simulink model "vdynblksskidpad_final"  (R2026b)
settings: Solver=ode23t  StopTime=inf  RelTol=5e-3
model workspace (MAT data in the model file):
  Eng : object (value not decoded)
  Nmtr = 11.5
  StartupTrim : object (value not decoded)
  SteerLim = 60
  TrackPoints = [-15 -12 -9 -6 -3 5.58745102111e-16 2.81978007367 5.36354042717 7.38228007367 8.67839071119 9.125 8.67839071119 ... (270 elements, 90x3)]
  Trans : object (value not decoded)
  Ts = 0.02
  VEH : object (value not decoded)
values from neighbouring files (symbols this model uses):
  n = size(e.Data,2)    [plot_skidpad_signals.m]
  z = tsMatrix(out.diagWheel.z)    [skidpad_settle_start.m]
symbols that are objects in the model workspace (value not decoded): Eng, StartupTrim, Trans, VEH
undefined symbols (not defined in the file or in its folder): BdyFrm, InertFrm, magnitude
libraries: autolibsharedcoupling x11, simulink x8, sim3dlib x7, autolibshareddiff x5, autolibutils x4, sim3dautolib x3, vehdynlibtirecommon x3, sharedtransform x3, vehdynlibdriver x2, vehdynlibsteering x2, vehdynlibeom x2, vehdynlibviscommon x2
(part 4 of 5)

== system vdynblksskidpad_final/Formula Student Vehicle/Simulink Physics - 7DOF/Powertrain & Driveline/Powertrain/4EM Powertrain/Mapped Motors ==
  BattVolt : Inport  Partition=on  PartitionDimension=1  PartitionWidth=1  PartitionOffset=0
  MtrSpd : Inport  Port=2  Partition=on  PartitionDimension=1  PartitionWidth=1  PartitionOffset=0
  TrqCmd : Inport  Port=3  Partition=on  PartitionDimension=1  PartitionWidth=1  PartitionOffset=0
  For Each : ForEach  DisableCoverage=on
  Mapped Motor : autolibmappedmotor/Mapped Motor  w_Tmax_bp_ext=[-800;-750;-375;0;375;750;800]  Tmax_w_V_ext=[0 0 0;0.07 0.07 0.07;0.08 0.08 0.08;0.09 0.09 0.09;0.08 0.08 0.08;0.07 0.07 0.07;0 0 0]  w_Tmin_bp_ext=[-800;-750;-375;0;375;750;800]  Tmin_w_V_ext=[0 0 0;-0.07 -0.07 -0.07;-0.08 -0.08 -0.08;-0.09 -0.09 -0.09;-0.08 -0.08 -0.08;-0.07 -0.07 -0.07;0 0 0]  port_config=Speed  param_by=Maximum torque and power  w_t=[0 954.93 1909.86 3819.72 4774.65 5729.58 7639.44 9549.30 11459.16 13369.02 15278.88 17188.74 19098.59 20000]*pi/30  T_t=[40 40 40 40 40 33.33 25.00 20.00 16.67 14.29 12.50 11.11 10.00 9.55]  torque_max=31.6  power_max=35000  SpreadsheetTqLimitsFileName=MotorCalibrationImportData.xlsx  Tmax_w_V=[0.09 0.09 0.09;0.08 0.08 0.08;0.07 0.07 0.07;0 0 0]  w_Tmax_bp=[ 0 375 750 800 ]  V_Tmax_bp=[500 750 900]  Tmin_w_V=[-0.09 -0.09 -0.09;-0.08 -0.08 -0.08;-0.07 -0.07 -0.07;0 0 0]  w_Tmin_bp=[ 0 375 750 800 ]  V_Tmin_bp=[500 750 900]  Tc=.02  param_loss=Single efficiency measurement  SpreadsheetLossFileName=MotorCalibrationImportData.xlsx  SpreadsheetEffFileName=MotorCalibrationImportData.xlsx  eff=96  w_eff=4000  T_eff=40  Piron=400  Pbase=0  w_eff_bp=[-8000 -4000 0 4000 8000]  T_eff_bp=[0 0.03 0.06 0.09]  Temp_eff_bp=[233.15 293.15 373.15]  V_eff_bp=[500 700 900]  losses_table=[1.49 1.67 2.21 3.10; 0.42 0.69 1.14 2.03; 0.06 0.24 0.78 1.68; 0.42 0.69 1.14 2.03; 1.49 1.67 2.21 3.10]  losses_table_3d=cat(3,1.05*[1.49 1.67 2.21 3.10; 0.42 0.69 1.14 2.03; 0.06 0.24 0.78 1.68; 0.42 0.69 1.14 2.03; 1.49 1.67 2.21 3.10],[1.49 1.67 2.21 3.10; 0.42 0.69 1.14 2.03; 0.06 0.24 0.78 1.68; 0.42 0.69 1.14 2.03; 1.49 1.67 2.21 3.10],1.03*[1.49 1.67 2.21 3.10; 0.42 0.69 1.14 2.03; 0.06 0.24 0.78 1.68; 0.42 0.69 1.14 2.03; 1.49 1.67 2.21 3.10])  losses_table_4d=cat(4,cat(3,[1.5645 0.441 0.063 0.441 1.5645;1.7535 0.7245 0.252 0.7245 1.7535;2.3205 1.197 0.819 1.197 2.3205;3.255 2.1315 1.764 2.1315 3.255],[1.5645 0.441 0.063 0.441 1.5645;1.7535 0.7245 0.252 0.7245 1.7535;2.3205 1.197 0.819 1.197 2.3205;3.255 2.1315 1.764 2.1315 3.255],[1.5645 0.441 0.063 0.441 1.5645;1.7535 0.7245 0.252 0.7245 1.7535;2.3205 1.197 0.819 1.197 2.3205;3.255 2.1315 1.764 2.1315 3.255]),cat(3,[1.49 0.42 0.06 0.42 1.49;1.67 0.69 0.24 0.69 1.67;2.21 1.14 0.78 1.14 2.21;3.1 2.03 1.68 2.03 3.1],[1.49 0.42 0.06 0.42 1.49;1.67 0.69 0.24 0.69 1.67;2.21 1.14 0.78 1.14 2.21;3.1 2.03 1.68 2.03 3.1],[1.49 0.42 0.06 0.42 1.49;1.67 0.69 0.24 0.69 1.67;2.21 1.14 0.78 1.14 2.21;3.1 2.03 1.68 2.03 3.1]),cat(3,[1.5347 0.4326 0.0618 0.4326 1.5347;1.7201 0.7107 0.2472 0.7107 1.7201;2.2763 1.1742 0.8034 1.1742 2.2763;3.193 2.0909 1.7304 2.0909 3.193],[1.5347 0.4326 0.0618 0.4326 1.5347;1.7201 0.7107 0.2472 0.7107 1.7201;2.2763 1.1742 0.8034 1.1742 2.2763;3.193 2.0909 1.7304 2.0909 3.193],[1.5347 0.4326 0.0618 0.4326 1.5347;1.7201 0.7107 0.2472 0.7107 1.7201;2.2763 1.1742 0.8034 1.1742 2.2763;3.193 2.0909 1.7304 2.0909 3.193]))  efficiency_table=[95 95 95 95; 95 95 95 95; 95 95 95 95; 95 95 95 95; 95 95 95 95]  efficiency_table_3d=cat(3,90*ones(5,4),95*ones(5,4),92*ones(5,4))  efficiency_table_4d=cat(4,cat(3,90*ones(5,4)',90*ones(5,4)',90*ones(5,4)'),cat(3,95*ones(5,4)',95*ones(5,4)',95*ones(5,4)'),cat(3,92*ones(5,4)',92*ones(5,4)',92*ones(5,4)'))  J=5e-6  b=1e-5  omega_o=0  T_t_extended=[0 15.4 17.6 20.9 17.6 15.4 0]  w_t_extended=[-8000 -7500 -3750 0 3750 7500 8000]  KLossIron=0  KLossCopper=0  x_w_eff_vec=[-8000 -4000 0 4000 8000]  x_T_eff_vec=[-0.09 -0.06 -0.03 0 0.03 0.06 0.09]  x_tmp_eff_vec=[233.15 293.15 373.15]  x_V_eff_vec=[500 700 900]  x_losses_mat=[3.1 2.21 1.67 1.49 1.67 2.21 3.1;2.03 1.14 0.69 0.42 0.69 1.14 2.03;1.68 0.78 0.24 0.06 0.24 0.78 1.68;2.03 1.14 0.69 0.42 0.69 1.14 2.03;3.1 2.21 1.67 1.49 1.67 2.21 3.1]  x_losses_mat_3d=cat(3,[3.255 2.3205 1.7535 1.5645 1.7535 2.3205 3.255;2.1315 1.197 0.7245 0.441 0.7245 1.197 2.1315;1.764 0.819 0.252 0.063 0.252 0.819 1.764;2.1315 1.197 0.7245 0.441 0.7245 1.197 2.1315;3.255 2.3205 1.7535 1.5645 1.7535 2.3205 3.255],[3.1 2.21 1.67 1.49 1.67 2.21 3.1;2.03 1.14 0.69 0.42 0.69 1.14 2.03;1.68 0.78 0.24 0.06 0.24 0.78 1.68;2.03 1.14 0.69 0.42 0.69 1.14 2.03;3.1 2.21 1.67 1.49 1.67 2.21 3.1],[3.193 2.2763 1.7201 1.5347 1.7201 2.2763 3.193;2.0909 1.1742 0.7107 0.4326 0.7107 1.1742 2.0909;1.7304 0.8034 0.2472 0.0618 0.2472 0.8034 1.7304;2.0909 1.1742 0.7107 0.4326 0.7107 1.1742 2.0909;3.193 2.2763 1.7201 1.5347 1.7201 2.2763 3.193])  x_losses_mat_4d=cat(4,cat(3,[1.5645 0.441 0.063 0.441 1.5645;1.7535 0.7245 0.252 0.7245 1.7535;2.3205 1.197 0.819 1.197 2.3205;3.255 2.1315 1.764 2.1315 3.255],[1.5645 0.441 0.063 0.441 1.5645;1.7535 0.7245 0.252 0.7245 1.7535;2.3205 1.197 0.819 1.197 2.3205;3.255 2.1315 1.764 2.1315 3.255],[1.5645 0.441 0.063 0.441 1.5645;1.7535 0.7245 0.252 0.7245 1.7535;2.3205 1.197 0.819 1.197 2.3205;3.255 2.1315 1.764 2.1315 3.255]),cat(3,[1.49 0.42 0.06 0.42 1.49;1.67 0.69 0.24 0.69 1.67;2.21 1.14 0.78 1.14 2.21;3.1 2.03 1.68 2.03 3.1],[1.49 0.42 0.06 0.42 1.49;1.67 0.69 0.24 0.69 1.67;2.21 1.14 0.78 1.14 2.21;3.1 2.03 1.68 2.03 3.1],[1.49 0.42 0.06 0.42 1.49;1.67 0.69 0.24 0.69 1.67;2.21 1.14 0.78 1.14 2.21;3.1 2.03 1.68 2.03 3.1]),cat(3,[1.5347 0.4326 0.0618 0.4326 1.5347;1.7201 0.7107 0.2472 0.7107 1.7201;2.2763 1.1742 0.8034 1.1742 2.2763;3.193 2.0909 1.7304 2.0909 3.193],[1.5347 0.4326 0.0618 0.4326 1.5347;1.7201 0.7107 0.2472 0.7107 1.7201;2.2763 1.1742 0.8034 1.1742 2.2763;3.193 2.0909 1.7304 2.0909 3.193],[1.5347 0.4326 0.0618 0.4326 1.5347;1.7201 0.7107 0.2472 0.7107 1.7201;2.2763 1.1742 0.8034 1.1742 2.2763;3.193 2.0909 1.7304 2.0909 3.193]))  CalLossMapData={}  CalLossWithTempMapData={}  aMode=2  RefBlkName='autolibmappedmotor/Mapped Motor'
      settings: LibrarySourceBlock=vdynlib/Powertrain/Propulsion/Mapped Motor
  Power and Torque Management : Subsystem
  Terminator : Terminator
  MtrTrq : Outport  ConcatenationDimension=1
  BattCurr : Outport  Port=2  ConcatenationDimension=1
  TrqLimCmd : Outport  Port=3  ConcatenationDimension=1
  wires:
  Mapped Motor/2 -> BattCurr/1
  TrqCmd/1 -> Power and Torque Management/2(TrqCmd)
  Mapped Motor/1 -> Terminator/1
  MtrSpd/1 -> Power and Torque Management/1(MtrSpd), Mapped Motor/2
  Mapped Motor/3 -> MtrTrq/1
  Power and Torque Management/1(TrqLimCmd) -> TrqLimCmd/1, Mapped Motor/3
  BattVolt/1 -> Mapped Motor/1

== system vdynblksskidpad_final/Formula Student Vehicle/Simulink Physics - 7DOF/Powertrain & Driveline/Powertrain/ICE Powertrain/Transmission ==
  EngTrq : Inport
  GearCmd : Inport  Port=2
  PropShftSpd : Inport  Port=3
  Ideal : Subsystem  VariantControl=0
  EngSpd : Outport  VectorParamsAs1DForOutWhenUnconnected=off
  Info : Outport  Port=2  VectorParamsAs1DForOutWhenUnconnected=off
  DrvShfTrq : Outport  Port=3  VectorParamsAs1DForOutWhenUnconnected=off

== system vdynblksskidpad_final/Visualization/3D Visualization/Enabled/3D Visualization/Ground Following/Annotations ==
  VehFdbk : Inport
  Disabled : Subsystem  VariantControl=annotOn==0
  Enabled : Subsystem  VariantControl=annotOn==1

== system vdynblksskidpad_final/Visualization/3D Visualization/Enabled/3D Visualization/Ground Following/Path ==
  VehFdbk : Inport
  Disabled : Subsystem  VariantControl=pathOn==0
  Enabled : Subsystem  VariantControl=pathOn==1

== system vdynblksskidpad_final/Visualization/3D Visualization/Enabled/3D Visualization/Physical Vehicle/Annotations ==
  VehFdbk : Inport
  Disabled : Subsystem  VariantControl=annotOn==0
  Enabled : Subsystem  VariantControl=annotOn==1

== system vdynblksskidpad_final/Visualization/3D Visualization/Enabled/3D Visualization/Physical Vehicle/Path ==
  VehFdbk : Inport
  Disabled : Subsystem  VariantControl=pathOn==0
  Enabled : Subsystem  VariantControl=pathOn==1

== system vdynblksskidpad_final/Visualization/3D Visualization/Enabled/3D Visualization/Simulation 3D Vehicle/Annotations ==
  VehFdbk : Inport
  Disabled : Subsystem  VariantControl=annotOn==0
  Enabled : Subsystem  VariantControl=annotOn==1

== system vdynblksskidpad_final/Visualization/3D Visualization/Enabled/3D Visualization/Simulation 3D Vehicle/Part Rotation Concatenation ==
  Body Roll : Inport
  Body Ptich : Inport  Port=2
  Body Yaw : Inport  Port=3
  WheelFrontLeft Pitch : Inport  Port=4
  WheelFrontRight Pitch : Inport  Port=5
  WheelRearLeft Pitch : Inport  Port=6
  WheelRearRight Ptich : Inport  Port=7
  WheelFrontLeft Roll : Inport  Port=8
  WheelFrontRight Roll : Inport  Port=9
  WheelRearLeft Roll : Inport  Port=10
  WheelRearRight Roll : Inport  Port=11
  WheelFrontLeft Yaw : Inport  Port=12
  WheelFrontRight Yaw : Inport  Port=13
  WheelRearLeft Yaw : Inport  Port=14
  WheelRearRight Yaw : Inport  Port=15
  AllParts : Concatenate  NumInputs=5  Mode=Multidimensional array
  Body : Concatenate  NumInputs=3  Mode=Multidimensional array  ConcatenateDimension=2
  WheelFrontLeft : Concatenate  NumInputs=3  Mode=Multidimensional array  ConcatenateDimension=2
  WheelFrontRight : Concatenate  NumInputs=3  Mode=Multidimensional array  ConcatenateDimension=2
  WheelRearLeft : Concatenate  NumInputs=3  Mode=Multidimensional array  ConcatenateDimension=2
  WheelRearRight : Concatenate  NumInputs=3  Mode=Multidimensional array  ConcatenateDimension=2
  ConcatOut : Outport  VectorParamsAs1DForOutWhenUnconnected=off
  wires:
  Body Yaw/1 -> Body/3
  WheelFrontLeft Yaw/1 -> WheelFrontLeft/3
  WheelFrontLeft/1 -> AllParts/2
  Body/1 -> AllParts/1
  WheelRearLeft/1 -> AllParts/4
  WheelFrontRight/1 -> AllParts/3
  WheelRearRight Yaw/1 -> WheelRearRight/3
  WheelRearLeft Yaw/1 -> WheelRearLeft/3
  AllParts/1 -> ConcatOut/1
  WheelRearRight/1 -> AllParts/5
  WheelFrontRight Yaw/1 -> WheelFrontRight/3
  Body Ptich/1 -> Body/2
  Body Roll/1 -> Body/1
  WheelFrontLeft Pitch/1 -> WheelFrontLeft/2
  WheelFrontLeft Roll/1 -> WheelFrontLeft/1
  WheelFrontRight Pitch/1 -> WheelFrontRight/2
  WheelFrontRight Roll/1 -> WheelFrontRight/1
  WheelRearLeft Pitch/1 -> WheelRearLeft/2
  WheelRearLeft Roll/1 -> WheelRearLeft/1
  WheelRearRight Ptich/1 -> WheelRearRight/2
  WheelRearRight Roll/1 -> WheelRearRight/1

== system vdynblksskidpad_final/Visualization/3D Visualization/Enabled/3D Visualization/Simulation 3D Vehicle/Part Translation Concatenation ==
  BodyX : Inport
  BodyY : Inport  Port=2
  BodyZ : Inport  Port=3
  WheelFrontLeftX : Inport  Port=4
  WheelFrontRightX : Inport  Port=5
  WheelRearLeftX : Inport  Port=6
  WheelRearRightX : Inport  Port=7
  WheelFrontLeftY : Inport  Port=8
  WheelFrontRightY : Inport  Port=9
  WheelRearLeftY : Inport  Port=10
  WheelRearRightY : Inport  Port=11
  WheelFrontLeftZ : Inport  Port=12
  WheelFrontRightZ : Inport  Port=13
  WheelRearLeftZ : Inport  Port=14
  WheelRearRightZ : Inport  Port=15
  AllParts : Concatenate  NumInputs=5  Mode=Multidimensional array
  Body : Concatenate  NumInputs=3  Mode=Multidimensional array  ConcatenateDimension=2
  WheelFrontLeft : Concatenate  NumInputs=3  Mode=Multidimensional array  ConcatenateDimension=2
  WheelFrontRight : Concatenate  NumInputs=3  Mode=Multidimensional array  ConcatenateDimension=2
  WheelRearLeft : Concatenate  NumInputs=3  Mode=Multidimensional array  ConcatenateDimension=2
  WheelRearRight : Concatenate  NumInputs=3  Mode=Multidimensional array  ConcatenateDimension=2
  ConcatOut : Outport  VectorParamsAs1DForOutWhenUnconnected=off
  wires:
  BodyX/1 -> Body/1
  BodyZ/1 -> Body/3
  WheelFrontLeftX/1 -> WheelFrontLeft/1
  WheelFrontLeftZ/1 -> WheelFrontLeft/3
  WheelFrontLeftY/1 -> WheelFrontLeft/2
  BodyY/1 -> Body/2
  WheelFrontLeft/1 -> AllParts/2
  WheelRearRightX/1 -> WheelRearRight/1
  Body/1 -> AllParts/1
  WheelRearLeft/1 -> AllParts/4
  WheelFrontRight/1 -> AllParts/3
  WheelRearRightZ/1 -> WheelRearRight/3
  WheelFrontRightY/1 -> WheelFrontRight/2
  WheelFrontRightX/1 -> WheelFrontRight/1
  WheelRearRightY/1 -> WheelRearRight/2
  WheelRearLeftZ/1 -> WheelRearLeft/3
  AllParts/1 -> ConcatOut/1
  WheelRearLeftY/1 -> WheelRearLeft/2
  WheelRearRight/1 -> AllParts/5
  WheelRearLeftX/1 -> WheelRearLeft/1
  WheelFrontRightZ/1 -> WheelFrontRight/3

== system vdynblksskidpad_final/Visualization/3D Visualization/Enabled/3D Visualization/Simulation 3D Vehicle/Path ==
  VehFdbk : Inport
  Disabled : Subsystem  VariantControl=pathOn==0
  Enabled : Subsystem  VariantControl=pathOn==1

== system vdynblksskidpad_final/Visualization/3D Visualization/Enabled/3D Visualization/Simulation 3D Vehicle/Scale ==
  Constant{1..12,17,32..33} (15 alike) : Constant  OutDataTypeStr=single
  PartConcatenation : Subsystem
  ScaleOut : Outport  VectorParamsAs1DForOutWhenUnconnected=off
  wires:
  Constant10/1 -> PartConcatenation/15(WheelRearRightZ)
  Constant9/1 -> PartConcatenation/14(WheelRearRightY)
  Constant11/1 -> PartConcatenation/13(WheelRearRightX)
  Constant7/1 -> PartConcatenation/12(WheelRearLeftZ)
  Constant6/1 -> PartConcatenation/11(WheelRearLeftY)
  Constant8/1 -> PartConcatenation/10(WheelRearLeftX)
  Constant4/1 -> PartConcatenation/9(WheelFrontRightZ)
  Constant3/1 -> PartConcatenation/8(WheelFrontRightY)
  Constant5/1 -> PartConcatenation/7(WheelFrontRightX)
  Constant2/1 -> PartConcatenation/6(WheelFrontLeftZ)
  Constant1/1 -> PartConcatenation/5(WheelFrontLeftY)
  Constant33/1 -> PartConcatenation/4(WheelFrontLeftX)
  Constant32/1 -> PartConcatenation/3(BodyZ)
  Constant17/1 -> PartConcatenation/2(BodyY)
  Constant12/1 -> PartConcatenation/1(BodyX)
  PartConcatenation/1(ConcatOut) -> ScaleOut/1

== system vdynblksskidpad_final/Formula Student Vehicle/Simulink Physics - 7DOF/Powertrain & Driveline/Powertrain/4EM Powertrain/Mapped Motors/Power and Torque Management ==
  MtrSpd : Inport
  TrqCmd : Inport  Port=2
  Abs1 : Abs  ZeroCross=off  SaturateOnIntegerOverflow=off
  Abs2 : Abs  ZeroCross=off  SaturateOnIntegerOverflow=off
  Divide1 : Product  Inputs=*/
  MaxPwr : Constant  Value=20e3
  Product : Product
  PwrLimCorner : Gain  Gain=2
  Saturation Dynamic : sl_discontinuities/Saturation Dynamic  OutMin=[]  OutMax=[]  OutDataTypeStr=Inherit: Same as second input  OutDataType=fixdt(1, 16)  OutScaling=2^-10  DoSatur=off
  Saturation2 : Saturate  UpperLimit=inf  LowerLimit=1  ZeroCross=off
  Saturation3 : Saturate  UpperLimit=40  LowerLimit=0  ZeroCross=off
  Subtract : Sum  Inputs=+-
  Transfer Fcn : TransferFcn  Denominator=[0.1 1]
  Unary Minus : UnaryMinus
  div0protect : autolibutils/div0protect - poly  thresh=1  ZeroCross=off  ZeroCross1=on  aMode=2
  TrqLimCmd : Outport
  wires:
  Product/1 -> Abs1/1
  MtrSpd/1 -> Product/2, Abs2/1
  MaxPwr/1 -> PwrLimCorner/1
  Abs1/1 -> Subtract/2
  Saturation2/1 -> Divide1/1  "PwrLim"
  Unary Minus/1 -> Saturation Dynamic/3
  Divide1/1 -> Saturation3/1
  Abs2/1 -> div0protect/1
  div0protect/1 -> Divide1/2
  TrqCmd/1 -> Saturation Dynamic/2
  Saturation3/1 -> Saturation Dynamic/1, Unary Minus/1  "AxlTrqLim"
  Subtract/1 -> Saturation2/1
  Saturation Dynamic/1 -> TrqLimCmd/1, Transfer Fcn/1
  Transfer Fcn/1 -> Product/1
  PwrLimCorner/1 -> Subtract/1

== system vdynblksskidpad_final/Formula Student Vehicle/Simulink Physics - 7DOF/Powertrain & Driveline/Powertrain/ICE Powertrain/Transmission/Ideal ==
  GearCmd : Inport
  EngTrq : Inport  Port=2
  PropShftSpd : Inport  Port=3
  Ideal Fixed Gear Transmission : autolibsharedtransfixedgear/Ideal Fixed Gear Transmission  VariantControl=0  TransEffModelPopup=Gear only  gearInterp=Linear point-slope  G=Trans.GearNums  Trq_bpts=[25, 50, 75, 100, 150, 200, 250]  omega_bpts=[52.4 78.5 105 131 157 183 209 262 314 419 524]  Temp_bpts=[313 358]  N=Trans.GearRatios  Jout=Trans.Inertias  bout=Trans.DampingCoeffs  eta=Trans.Efficiencies  eta_tbl=reshape([0.53 0.71 0.77 0.79 0.82 0.82 0.82 0.5 0.7 0.77 0.79 0.82 0.82 0.82 0.54 0.72 0.78 0.81 0.83 0.82 0.82 0.56 0.73 0.79 0.81 0.84 0.82 0.82 0.58 0.74 0.79 0.82 0.84 0.82 0.82 0.57 0.74 0.79 0.82 0.84 0.82 0.82 0.58 0.74 0.79 0.82 0.84 0.82 0.82 0.58 0.74 0.79 0.82 0.84 0.82 0.82 0.57 0.74 0.8 0.82 0.85 0.82 0.82 0.55 0.73 0.78 0.81 0.84 0.82 0.82 0.51 0.71 0.77 0.81 0.84 0.82 0.82 0.53 0.71 0.77 0.79 0.82 0.82 0.82 0.5 0.7 0.77 0.79 0.82 0.82 0.82 0.54 0.72 0.78 0.81 0.83 0.82 0.82 0.56 0.73 0.79 0.81 0.84 0.82 0.82 0.58 0.74 0.79 0.82 0.84 0.82 0.82 0.57 0.74 0.79 0.82 0.84 0.82 0.82 0.58 0.74 0.79 0.82 0.84 0.82 0.82 0.58 0.74 0.79 0.82 0.84 0.82 0.82 0.57 0.74 0.8 0.82 0.85 0.82 0.82 0.55 0.73 0.78 0.81 0.84 0.82 0.82 0.51 0.71 0.77 0.81 0.84 0.82 0.82 0.53 0.71 0.77 0.79 0.82 0.82 0.82 0.5 0.7 0.77 0.79 0.82 0.82 0.82 0.54 0.72 0.78 0.81 0.83 0.82 0.82 0.56 0.73 0.79 0.81 0.84 0.82 0.82 0.58 0.74 0.79 0.82 0.84 0.82 0.82 0.57 0.74 0.79 0.82 0.84 0.82 0.82 0.58 0.74 0.79 0.82 0.84 0.82 0.82 0.58 0.74 0.79 0.82 0.84 0.82 0.82 0.57 0.74 0.8 0.82 0.85 0.82 0.82 0.55 0.73 0.78 0.81 0.84 0.82 0.82 0.51 0.71 0.77 0.81 0.84 0.82 0.82 0.7 0.79 0.82 0.83 0.84 0.84 0.84 0.63 0.76 0.8 0.82 0.83 0.84 0.84 0.58 0.74 0.79 0.81 0.83 0.84 0.84 0.58 0.74 0.79 0.81 0.83 0.84 0.84 0.58 0.74 0.79 0.81 0.84 0.84 0.84 0.57 0.73 0.78 0.81 0.84 0.85 0.84 0.57 0.73 0.79 0.81 0.84 0.85 0.84 0.56 0.73 0.78 0.81 0.83 0.85 0.84 0.55 0.73 0.78 0.81 0.84 0.85 0.84 0.52 0.71 0.77 0.8 0.83 0.85 0.84 0.48 0.69 0.76 0.79 0.83 0.84 0.84 0.64 0.76 0.8 0.81 0.83 0.84 0.84 0.56 0.73 0.78 0.8 0.83 0.84 0.84 0.54 0.71 0.77 0.8 0.82 0.84 0.84 0.53 0.71 0.77 0.8 0.83 0.84 0.84 0.51 0.71 0.77 0.8 0.83 0.84 0.85 0.52 0.7 0.77 0.8 0.83 0.84 0.85 0.51 0.71 0.76 0.79 0.83 0.84 0.85 0.5 0.69 0.76 0.79 0.82 0.84 0.85 0.45 0.68 0.75 0.78 0.82 0.84 0.85 0.43 0.67 0.74 0.78 0.81 0.83 0.84 0.38 0.63 0.71 0.75 0.8 0.82 0.83 0.65 0.79 0.84 0.85 0.88 0.89 0.89 0.56 0.75 0.81 0.83 0.86 0.88 0.89 0.52 0.72 0.79 0.83 0.86 0.88 0.88 0.51 0.72 0.79 0.83 0.86 0.88 0.89 0.49 0.71 0.78 0.82 0.86 0.88 0.89 0.47 0.7 0.78 0.82 0.86 0.87 0.88 0.45 0.69 0.77 0.81 0.85 0.87 0.88 0.4 0.67 0.75 0.8 0.84 0.86 0.88 0.3 0.64 0.73 0.78 0.83 0.86 0.87 0.17 0.55 0.67 0.73 0.8 0.83 0.85 0.089 0.45 0.61 0.69 0.77 0.81 0.83 0.61 0.75 0.82 0.84 0.87 0.87 0.88 0.54 0.73 0.8 0.82 0.86 0.87 0.88 0.51 0.71 0.79 0.82 0.86 0.87 0.88 0.52 0.72 0.79 0.82 0.86 0.87 0.89 0.52 0.72 0.8 0.83 0.86 0.88 0.89 0.53 0.72 0.79 0.82 0.86 0.87 0.89 0.5 0.7 0.78 0.82 0.86 0.88 0.88 0.46 0.69 0.77 0.81 0.85 0.87 0.88 0.4 0.67 0.75 0.8 0.83 0.86 0.88 0.33 0.64 0.73 0.78 0.83 0.85 0.87 0.33 0.64 0.73 0.78 0.83 0.85 0.87 0.78 0.85 0.87 0.88 0.89 0.89 0.89 0.73 0.83 0.86 0.88 0.89 0.89 0.89 0.72 0.83 0.86 0.88 0.89 0.89 0.89 0.72 0.83 0.87 0.89 0.9 0.89 0.89 0.72 0.83 0.87 0.88 0.9 0.89 0.89 0.71 0.83 0.87 0.88 0.9 0.89 0.89 0.71 0.83 0.86 0.88 0.9 0.89 0.89 0.7 0.82 0.86 0.88 0.9 0.89 0.89 0.69 0.82 0.86 0.88 0.9 0.89 0.89 0.67 0.81 0.86 0.88 0.9 0.89 0.89 0.63 0.79 0.85 0.87 0.89 0.89 0.89 0.78 0.85 0.87 0.88 0.89 0.89 0.89 0.73 0.83 0.86 0.88 0.89 0.89 0.89 0.72 0.83 0.86 0.88 0.89 0.89 0.89 0.72 0.83 0.87 0.89 0.9 0.89 0.89 0.72 0.83 0.87 0.88 0.9 0.89 0.89 0.71 0.83 0.87 0.88 0.9 0.89 0.89 0.71 0.83 0.86 0.88 0.9 0.89 0.89 0.7 0.82 0.86 0.88 0.9 0.89 0.89 0.69 0.82 0.86 0.88 0.9 0.89 0.89 0.67 0.81 0.86 0.88 0.9 0.89 0.89 0.63 0.79 0.85 0.87 0.89 0.89 0.89 0.78 0.85 0.87 0.88 0.89 0.89 0.89 0.73 0.83 0.86 0.88 0.89 0.89 0.89 0.72 0.83 0.86 0.88 0.89 0.89 0.89 0.72 0.83 0.87 0.89 0.9 0.89 0.89 0.72 0.83 0.87 0.88 0.9 0.89 0.89 0.71 0.83 0.87 0.88 0.9 0.89 0.89 0.71 0.83 0.86 0.88 0.9 0.89 0.89 0.7 0.82 0.86 0.88 0.9 0.89 0.89 0.69 0.82 0.86 0.88 0.9 0.89 0.89 0.67 0.81 0.86 0.88 0.9 0.89 0.89 0.63 0.79 0.85 0.87 0.89 0.89 0.89 0.82 0.87 0.88 0.89 0.89 0.89 0.89 0.81 0.87 0.89 0.89 0.9 0.9 0.89 0.76 0.85 0.87 0.89 0.9 0.89 0.89 0.72 0.83 0.86 0.88 0.89 0.89 0.89 0.72 0.83 0.86 0.88 0.89 0.9 0.89 0.71 0.82 0.86 0.88 0.89 0.9 ...(+1314 chars))  G_o=0  omega_o=0  omegaN_o=0  tau_s=Trans.ShiftTau  maxAbsSpd=5e3  aMode=2
      settings: LibrarySourceBlock=vdynlib/Powertrain/Transmission/Ideal Fixed Gear Transmission
  Prop Shaft : autolibsharedcoupling/Torsional Compliance  port_config=Simulink  extInfo=off  k=5e3  b=10  theta_o=0  domega_o=0  omega_c=100  blkID=0  aMode=2
      settings: LibrarySourceBlock=vdynlib/Powertrain/Drivetrain/Couplings/Torsional Compliance
  Unit Conversion : UnitConversion
  Info : Outport  VectorParamsAs1DForOutWhenUnconnected=off
  EngSpd : Outport  Port=2  VectorParamsAs1DForOutWhenUnconnected=off
  DrvShfTrq : Outport  Port=3  VectorParamsAs1DForOutWhenUnconnected=off
  wires:
  Ideal Fixed Gear Transmission/2 -> Unit Conversion/1
  GearCmd/1 -> Ideal Fixed Gear Transmission/1
  Ideal Fixed Gear Transmission/1 -> Info/1
  PropShftSpd/1 -> Prop Shaft/2
  Ideal Fixed Gear Transmission/3 -> Prop Shaft/1
  Prop Shaft/2 -> DrvShfTrq/1
  Prop Shaft/1 -> Ideal Fixed Gear Transmission/3
  EngTrq/1 -> Ideal Fixed Gear Transmission/2
  Unit Conversion/1 -> EngSpd/1

== system vdynblksskidpad_final/Visualization/3D Visualization/Enabled/3D Visualization/Ground Following/Annotations/Disabled ==

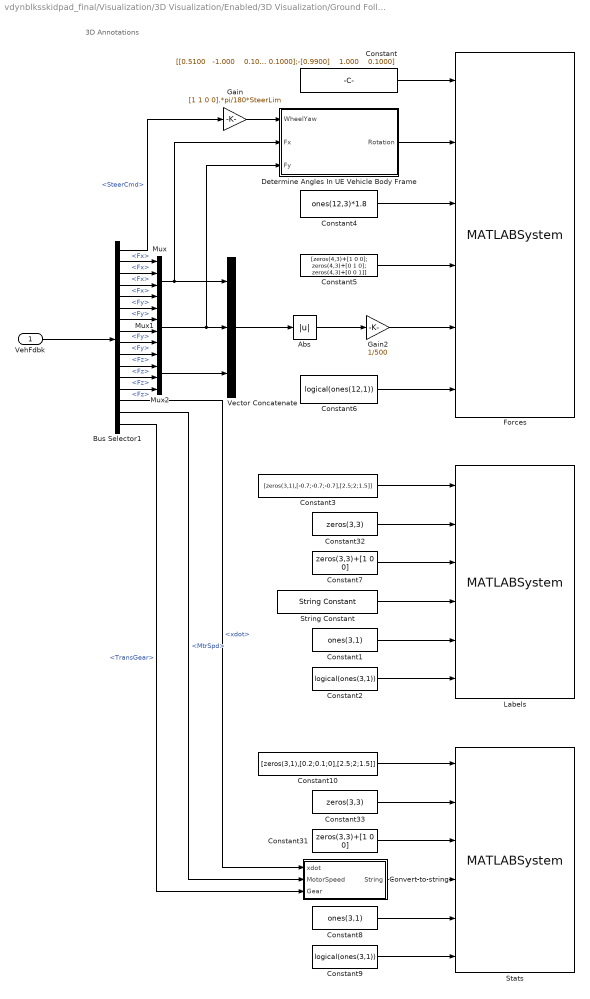
== system vdynblksskidpad_final/Visualization/3D Visualization/Enabled/3D Visualization/Ground Following/Annotations/Enabled ==
  note: 3D Annotations
  VehFdbk : Inport
  Abs : Abs  ZeroCross=off  SaturateOnIntegerOverflow=off
  Bus Selector1 : BusSelector  OutputSignals=Driver.SteerCmd,VehFdbk.BdyFrm.Forces.Tires.FrntTires.Lft.Fx,VehFdbk.BdyFrm.Forces.Tires.FrntTires.Rght.Fx,VehFdbk.BdyFrm.Forces.Tires.RearTires.Lft.Fx,VehFdbk.BdyFrm.Forces.Tires.RearTires.Rght.Fx,VehFdbk.BdyFrm.Forces.Tires.FrntTires.Lft.Fy,VehFdbk.BdyFrm.Forces.Tires.FrntTires.Rght.Fy,VehFdbk.BdyFrm.Forces.Tires.RearTires.Lft.Fy,VehFdbk.BdyFrm.Forces.Tires.RearTires.Rght.Fy,VehFdbk.BdyFrm.Forces.Tires.FrntTires.Lft.Fz,VehFdbk.BdyFrm.Forces.Tires.FrntTires.Rght.Fz,VehFdbk.BdyFrm.Forces.Tires.RearTires.Lft.Fz,VehFdbk.BdyFrm.Forces.Tires.RearTires.Rght.Fz,VehFdbk.BdyFrm.Cg.Vel.xdot,VehFdbk.Mtr.MtrSpd,VehFdbk.Trans.TransGear
  Constant : Constant  Value="[[0.5100   -1.000    0.1000];[0.5100    1.000    0.1000];[-0.9900   -1.000    0.1000];[-0.9900    1.000    0.1000];[0.5100   -1.000    0.1000];[0.5100    1.000    0.1000];[-0.9900   -1.000    0.1000];[-0.9900    1.000    0.1000];[0.5100   -1.000    0.1000];[0.5100    1.000    0.1000];[-0.9900   -1.000    0.1000];-[0.9900]    1.000    0.1000]"
  Constant1 : Constant  Value=ones(3,1)
  Constant10 : Constant  Value=[zeros(3,1),[0.2;0.1;0],[2.5;2;1.5]]
  Constant2 : Constant  Value=logical(ones(3,1))
  Constant3 : Constant  Value=[zeros(3,1),[-0.7;-0.7;-0.7],[2.5;2;1.5]]
  Constant31 : Constant  Value=zeros(3,3)+[1 0 0]
  Constant32 : Constant  Value=zeros(3,3)
  Constant33 : Constant  Value=zeros(3,3)
  Constant4 : Constant  Value=ones(12,3)*1.8
  Constant5 : Constant  Value=[zeros(4,3)+[1 0 0]; zeros(4,3)+[0 1 0]; zeros(4,3)+[0 0 1]]
  Constant6 : Constant  Value=logical(ones(12,1))
  Constant7 : Constant  Value=zeros(3,3)+[1 0 0]
  Constant8 : Constant  Value=ones(3,1)
  Constant9 : Constant  Value=logical(ones(3,1))
  Convert to string : Subsystem
  Determine Angles In UE Vehicle Body Frame : Subsystem
  Forces : MATLABSystem  Priority=-1  System=Simulation3DAnnotation  InitialPos="[[0.5100   -1.000    0.1000];[0.5100    1.000    0.1000];[-0.9900   -1.000    0.1000];[-0.9900    1.000    0.1000];[0.5100   -1.000    0.1000];[0.5100    1.000    0.1000];[-0.9900   -1.000    0.1000];[-0.9900    1.000    0.1000];[0.5100   -1.000    0.1000];[0.5100    1.000    0.1000];[-0.9900   -1.000    0.1000];-[0.9900]    1.000    0.1000]"  InitialRot=[zeros(4,3);[zeros(4,3)+[0 0 pi/2]];[zeros(4,3)+[0 pi/2 0]]]  InitialScale=zeros(12,3)  ActorTag=AnnotationActor1  ParentActor=SimulinkVehicle2  Color=[zeros(4,3)+[1 0 0]; zeros(4,3)+[0 1 0]; zeros(4,3)+[0 0 1]]  Length=zeros(12,1)  FontScale=1  IsHidden=logical(zeros(12,1))  SampleTime=Ts
      mask Type: Simulation3DAnnotation
  Gain : Gain  Gain=[1 1 0 0].*pi/180*SteerLim
  Gain2 : Gain  Gain=1/500
  Labels : MATLABSystem  Priority=-1  System=Simulation3DAnnotation  InitialPos=[zeros(3,1),[-0.7;-0.7;-0.7],[2.5;2;1.5]]  InitialRot=zeros(3,3)  InitialScale=zeros(3,3)  ActorTag=AnnotationActor2  ParentActor=SimulinkVehicle2  Color=zeros(3,3)+[1 0 0]  Length=1  String=Velocity\n Engine\n Gear  FontScale=ones(3,1)  IsHidden=logical(ones(3,1))  SampleTime=Ts
      mask Type: Simulation3DAnnotation
  Mux : Mux
  Mux1 : Mux
  Mux2 : Mux
  Stats : MATLABSystem  Priority=-1  System=Simulation3DAnnotation  InitialPos=[zeros(3,1),[0.2;0.1;0],[2.5;2;1.5]]  InitialRot=zeros(3,3)  InitialScale=zeros(3,3)  ActorTag=AnnotationActor3  ParentActor=SimulinkVehicle2  Color=zeros(3,3)+[1 0 0]  Length=1  String=00 km/h\n 0000 RPM\n 0  FontScale=ones(3,1)  IsHidden=logical(ones(3,1))  SampleTime=Ts
      mask Type: Simulation3DAnnotation
  String Constant : StringConstant  String="\"Velocity\\n Engine\\n Gear\""
  Vector Concatenate : Concatenate  NumInputs=3
  wires:
  VehFdbk/1 -> Bus Selector1/1
  Determine Angles In UE Vehicle Body Frame/1(Rotation) -> Forces/2
  Mux/1 -> Vector Concatenate/1, Determine Angles In UE Vehicle Body Frame/2(Fx)
  Mux1/1 -> Determine Angles In UE Vehicle Body Frame/3(Fy), Vector Concatenate/2
  Bus Selector1/1 -> Gain/1  "<SteerCmd>"
  Convert to string/1(String) -> Stats/4
  String Constant/1 -> Labels/4
  Constant33/1 -> Stats/2
  Constant31/1 -> Stats/3
  Constant8/1 -> Stats/5
  Constant9/1 -> Stats/6
  Constant32/1 -> Labels/2
  Constant3/1 -> Labels/1
  Constant7/1 -> Labels/3
  Constant1/1 -> Labels/5
  Constant2/1 -> Labels/6
  Constant10/1 -> Stats/1
  Constant/1 -> Forces/1
  Mux2/1 -> Vector Concatenate/3
  Abs/1 -> Gain2/1
  Vector Concatenate/1 -> Abs/1
  Gain2/1 -> Forces/5
  Constant4/1 -> Forces/3
  Constant6/1 -> Forces/6
  Constant5/1 -> Forces/4
  Gain/1 -> Determine Angles In UE Vehicle Body Frame/1(WheelYaw)
  Bus Selector1/2 -> Mux/1  "<Fx>"
  Bus Selector1/3 -> Mux/2  "<Fx>"
  Bus Selector1/4 -> Mux/3  "<Fx>"
  Bus Selector1/5 -> Mux/4  "<Fx>"
  Bus Selector1/6 -> Mux1/1  "<Fy>"
  Bus Selector1/7 -> Mux1/2  "<Fy>"
  Bus Selector1/8 -> Mux1/3  "<Fy>"
  Bus Selector1/9 -> Mux1/4  "<Fy>"
  Bus Selector1/10 -> Mux2/1  "<Fz>"
  Bus Selector1/11 -> Mux2/2  "<Fz>"
  Bus Selector1/12 -> Mux2/3  "<Fz>"
  Bus Selector1/13 -> Mux2/4  "<Fz>"
  Bus Selector1/14 -> Convert to string/1(xdot)  "<xdot>"
  Bus Selector1/15 -> Convert to string/2(MotorSpeed)  "<MtrSpd>"
  Bus Selector1/16 -> Convert to string/3(Gear)  "<TransGear>"

== system vdynblksskidpad_final/Visualization/3D Visualization/Enabled/3D Visualization/Ground Following/Path/Disabled ==

== system vdynblksskidpad_final/Visualization/3D Visualization/Enabled/3D Visualization/Ground Following/Path/Enabled ==
  VehFdbk : Inport
  Bus Selector : BusSelector  OutputSignals=VehFdbk.BdyFrm.Cg.Acc.ax,VehFdbk.BdyFrm.Cg.Acc.ay
  Constant5 : Constant
  Constant6 : Constant  Value=0
  Hypot : Math  Operator=hypot
  Saturation : Saturate  UpperLimit=1  LowerLimit=0  ZeroCross=off
  Simulation 3D Actor : sim3dlib/Simulation 3D Actor  ActorName=GrndVehPath  ParentName=Scene Origin  Operation=Create at setup  InitScriptText=|  SampleTime=Ts*5  Translation=[0 0 0]  Rotation=[0 0 0]  Scale=[1 1 1]  InputsText=PathMarker.Color  aMode=5  ActorTag=GrndVehPath  ActorType=Sim3dActor  ID=C
      | path1 = sim3d.graphics.PathMarker("ActorName", "PathMarker", ControlActorName="SimulinkVehicle3");
      | path1.MarkersSize = ones(1,3)*0.25;
      | path1.Color = [0 0 1];
      | World.add(path1,Actor);
  Sum1 : Sum  Inputs=|++
  Terminator4 : Terminator
  Unary Minus : UnaryMinus
  Vector Concatenate : Concatenate  NumInputs=3  Mode=Multidimensional array  ConcatenateDimension=2
  wires:
  Hypot/1 -> Saturation/1
  Saturation/1 -> Unary Minus/1, Vector Concatenate/1
  Constant5/1 -> Sum1/2
  Simulation 3D Actor/1 -> Terminator4/1
  Sum1/1 -> Vector Concatenate/3
  Unary Minus/1 -> Sum1/1
  Constant6/1 -> Vector Concatenate/2
  VehFdbk/1 -> Bus Selector/1
  Bus Selector/2 -> Hypot/2  "<ay>"
  Bus Selector/1 -> Hypot/1  "<ax>"
  Vector Concatenate/1 -> Simulation 3D Actor/1

== system vdynblksskidpad_final/Visualization/3D Visualization/Enabled/3D Visualization/Physical Vehicle/Annotations/Disabled ==

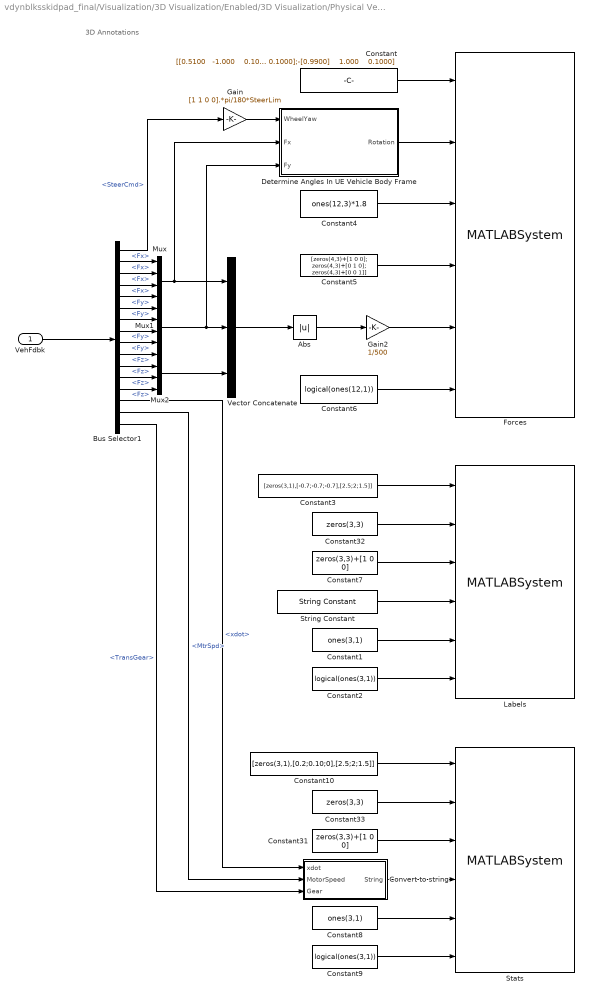
== system vdynblksskidpad_final/Visualization/3D Visualization/Enabled/3D Visualization/Physical Vehicle/Annotations/Enabled ==
  note: 3D Annotations
  VehFdbk : Inport
  Abs : Abs  ZeroCross=off  SaturateOnIntegerOverflow=off
  Bus Selector1 : BusSelector  OutputSignals=Driver.SteerCmd,VehFdbk.BdyFrm.Forces.Tires.FrntTires.Lft.Fx,VehFdbk.BdyFrm.Forces.Tires.FrntTires.Rght.Fx,VehFdbk.BdyFrm.Forces.Tires.RearTires.Lft.Fx,VehFdbk.BdyFrm.Forces.Tires.RearTires.Rght.Fx,VehFdbk.BdyFrm.Forces.Tires.FrntTires.Lft.Fy,VehFdbk.BdyFrm.Forces.Tires.FrntTires.Rght.Fy,VehFdbk.BdyFrm.Forces.Tires.RearTires.Lft.Fy,VehFdbk.BdyFrm.Forces.Tires.RearTires.Rght.Fy,VehFdbk.BdyFrm.Forces.Tires.FrntTires.Lft.Fz,VehFdbk.BdyFrm.Forces.Tires.FrntTires.Rght.Fz,VehFdbk.BdyFrm.Forces.Tires.RearTires.Lft.Fz,VehFdbk.BdyFrm.Forces.Tires.RearTires.Rght.Fz,VehFdbk.BdyFrm.Cg.Vel.xdot,VehFdbk.Mtr.MtrSpd,VehFdbk.Trans.TransGear
  Constant : Constant  Value="[[0.5100   -1.000    0.1000];[0.5100    1.000    0.1000];[-0.9900   -1.000    0.1000];[-0.9900    1.000    0.1000];[0.5100   -1.000    0.1000];[0.5100    1.000    0.1000];[-0.9900   -1.000    0.1000];[-0.9900    1.000    0.1000];[0.5100   -1.000    0.1000];[0.5100    1.000    0.1000];[-0.9900   -1.000    0.1000];-[0.9900]    1.000    0.1000]"
  Constant1 : Constant  Value=ones(3,1)
  Constant10 : Constant  Value=[zeros(3,1),[0.2;0.10;0],[2.5;2;1.5]]
  Constant2 : Constant  Value=logical(ones(3,1))
  Constant3 : Constant  Value=[zeros(3,1),[-0.7;-0.7;-0.7],[2.5;2;1.5]]
  Constant31 : Constant  Value=zeros(3,3)+[1 0 0]
  Constant32 : Constant  Value=zeros(3,3)
  Constant33 : Constant  Value=zeros(3,3)
  Constant4 : Constant  Value=ones(12,3)*1.8
  Constant5 : Constant  Value=[zeros(4,3)+[1 0 0]; zeros(4,3)+[0 1 0]; zeros(4,3)+[0 0 1]]
  Constant6 : Constant  Value=logical(ones(12,1))
  Constant7 : Constant  Value=zeros(3,3)+[1 0 0]
  Constant8 : Constant  Value=ones(3,1)
  Constant9 : Constant  Value=logical(ones(3,1))
  Convert to string : Subsystem
  Determine Angles In UE Vehicle Body Frame : Subsystem
  Forces : MATLABSystem  Priority=-1  System=Simulation3DAnnotation  InitialPos="[[0.5100   -1.000    0.1000];[0.5100    1.000    0.1000];[-0.9900   -1.000    0.1000];[-0.9900    1.000    0.1000];[0.5100   -1.000    0.1000];[0.5100    1.000    0.1000];[-0.9900   -1.000    0.1000];[-0.9900    1.000    0.1000];[0.5100   -1.000    0.1000];[0.5100    1.000    0.1000];[-0.9900   -1.000    0.1000];-[0.9900]    1.000    0.1000]"  InitialRot=[zeros(4,3);[zeros(4,3)+[0 0 pi/2]];[zeros(4,3)+[0 pi/2 0]]]  InitialScale=zeros(12,3)  ActorTag=AnnotationActor1  ParentActor=SimulinkVehicle2  Color=[zeros(4,3)+[1 0 0]; zeros(4,3)+[0 1 0]; zeros(4,3)+[0 0 1]]  Length=zeros(12,1)  FontScale=1  IsHidden=logical(zeros(12,1))  SampleTime=Ts
      mask Type: Simulation3DAnnotation
  Gain : Gain  Gain=[1 1 0 0].*pi/180*SteerLim
  Gain2 : Gain  Gain=1/500
  Labels : MATLABSystem  Priority=-1  System=Simulation3DAnnotation  InitialPos=[zeros(3,1),[-0.7;-0.7;-0.7],[2.5;2;1.5]]  InitialRot=zeros(3,3)  InitialScale=zeros(3,3)  ActorTag=AnnotationActor2  ParentActor=SimulinkVehicle2  Color=zeros(3,3)+[1 0 0]  Length=1  String=Velocity\n Engine\n Gear  FontScale=ones(3,1)  IsHidden=logical(ones(3,1))  SampleTime=Ts
      mask Type: Simulation3DAnnotation
  Mux : Mux
  Mux1 : Mux
  Mux2 : Mux
  Stats : MATLABSystem  Priority=-1  System=Simulation3DAnnotation  InitialPos=[zeros(3,1),[0.2;0.1;0.0],[2.5;2;1.5]]  InitialRot=zeros(3,3)  InitialScale=zeros(3,3)  ActorTag=AnnotationActor3  ParentActor=SimulinkVehicle2  Color=zeros(3,3)+[1 0 0]  Length=1  String=00 km/h\n 0000 RPM\n 0  FontScale=ones(3,1)  IsHidden=logical(ones(3,1))  SampleTime=Ts
      mask Type: Simulation3DAnnotation
  String Constant : StringConstant  String="\"Velocity\\n Engine\\n Gear\""
  Vector Concatenate : Concatenate  NumInputs=3
  wires:
  VehFdbk/1 -> Bus Selector1/1
  Determine Angles In UE Vehicle Body Frame/1(Rotation) -> Forces/2
  Mux/1 -> Vector Concatenate/1, Determine Angles In UE Vehicle Body Frame/2(Fx)
  Mux1/1 -> Determine Angles In UE Vehicle Body Frame/3(Fy), Vector Concatenate/2
  Bus Selector1/1 -> Gain/1  "<SteerCmd>"
  Convert to string/1(String) -> Stats/4
  String Constant/1 -> Labels/4
  Constant33/1 -> Stats/2
  Constant31/1 -> Stats/3
  Constant8/1 -> Stats/5
  Constant9/1 -> Stats/6
  Constant32/1 -> Labels/2
  Constant3/1 -> Labels/1
  Constant7/1 -> Labels/3
  Constant1/1 -> Labels/5
  Constant2/1 -> Labels/6
  Constant10/1 -> Stats/1
  Constant/1 -> Forces/1
  Mux2/1 -> Vector Concatenate/3
  Abs/1 -> Gain2/1
  Vector Concatenate/1 -> Abs/1
  Gain2/1 -> Forces/5
  Constant4/1 -> Forces/3
  Constant6/1 -> Forces/6
  Constant5/1 -> Forces/4
  Gain/1 -> Determine Angles In UE Vehicle Body Frame/1(WheelYaw)
  Bus Selector1/2 -> Mux/1  "<Fx>"
  Bus Selector1/3 -> Mux/2  "<Fx>"
  Bus Selector1/4 -> Mux/3  "<Fx>"
  Bus Selector1/5 -> Mux/4  "<Fx>"
  Bus Selector1/6 -> Mux1/1  "<Fy>"
  Bus Selector1/7 -> Mux1/2  "<Fy>"
  Bus Selector1/8 -> Mux1/3  "<Fy>"
  Bus Selector1/9 -> Mux1/4  "<Fy>"
  Bus Selector1/10 -> Mux2/1  "<Fz>"
  Bus Selector1/11 -> Mux2/2  "<Fz>"
  Bus Selector1/12 -> Mux2/3  "<Fz>"
  Bus Selector1/13 -> Mux2/4  "<Fz>"
  Bus Selector1/14 -> Convert to string/1(xdot)  "<xdot>"
  Bus Selector1/15 -> Convert to string/2(MotorSpeed)  "<MtrSpd>"
  Bus Selector1/16 -> Convert to string/3(Gear)  "<TransGear>"

== system vdynblksskidpad_final/Visualization/3D Visualization/Enabled/3D Visualization/Physical Vehicle/Path/Disabled ==

== system vdynblksskidpad_final/Visualization/3D Visualization/Enabled/3D Visualization/Physical Vehicle/Path/Enabled ==
  VehFdbk : Inport
  Bus Selector : BusSelector  OutputSignals=VehFdbk.BdyFrm.Cg.Acc.ax,VehFdbk.BdyFrm.Cg.Acc.ay
  Constant5 : Constant
  Constant6 : Constant  Value=0
  Hypot : Math  Operator=hypot
  Saturation : Saturate  UpperLimit=1  LowerLimit=0  ZeroCross=off
  Simulation 3D Actor : sim3dlib/Simulation 3D Actor  ActorName=GamePhysVehPath  ParentName=Scene Origin  Operation=Create at setup  InitScriptText=|  SampleTime=Ts*5  Translation=[0 0 0]  Rotation=[0 0 0]  Scale=[1 1 1]  InputsText=PathMarker.Color  aMode=5  ActorTag=GamePhysVehPath  ActorType=Sim3dActor  ID=C
      | path1 = sim3d.graphics.PathMarker("ActorName", "PathMarker", ControlActorName="SimulinkVehicle2");
      | path1.MarkersSize = ones(1,3)*0.25;
      | path1.Color = [0 0 1];
      | World.add(path1,Actor);
  Sum1 : Sum  Inputs=|++
  Terminator4 : Terminator
  Unary Minus : UnaryMinus
  Vector Concatenate : Concatenate  NumInputs=3  Mode=Multidimensional array  ConcatenateDimension=2
  wires:
  Hypot/1 -> Saturation/1
  Saturation/1 -> Unary Minus/1, Vector Concatenate/1
  Constant5/1 -> Sum1/2
  Simulation 3D Actor/1 -> Terminator4/1
  Sum1/1 -> Vector Concatenate/3
  Unary Minus/1 -> Sum1/1
  Constant6/1 -> Vector Concatenate/2
  VehFdbk/1 -> Bus Selector/1
  Bus Selector/2 -> Hypot/2  "<ay>"
  Bus Selector/1 -> Hypot/1  "<ax>"
  Vector Concatenate/1 -> Simulation 3D Actor/1

== system vdynblksskidpad_final/Visualization/3D Visualization/Enabled/3D Visualization/Simulation 3D Vehicle/Annotations/Disabled ==

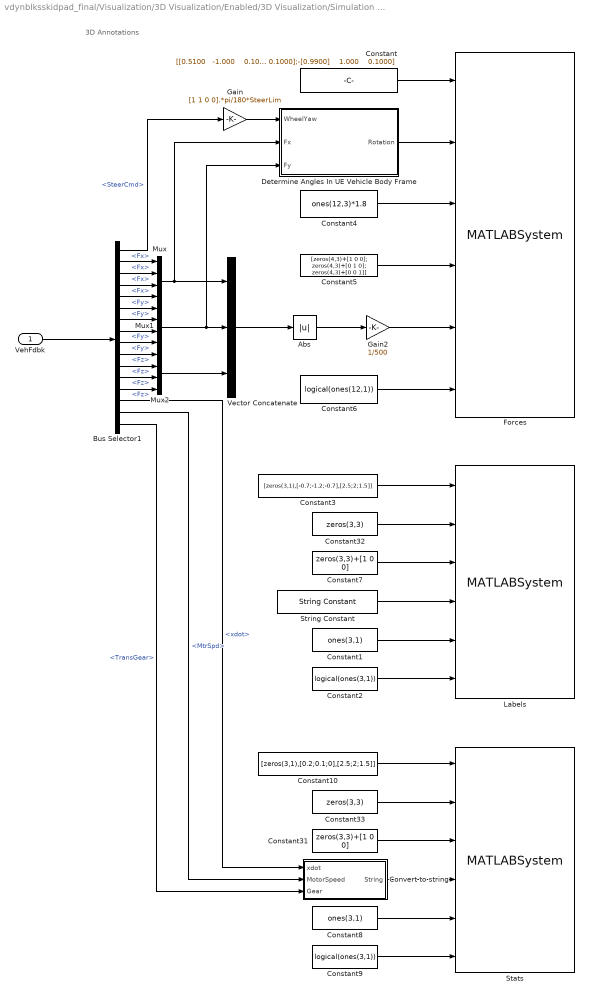
== system vdynblksskidpad_final/Visualization/3D Visualization/Enabled/3D Visualization/Simulation 3D Vehicle/Annotations/Enabled ==
  note: 3D Annotations
  VehFdbk : Inport
  Abs : Abs  ZeroCross=off  SaturateOnIntegerOverflow=off
  Bus Selector1 : BusSelector  OutputSignals=Driver.SteerCmd,VehFdbk.BdyFrm.Forces.Tires.FrntTires.Lft.Fx,VehFdbk.BdyFrm.Forces.Tires.FrntTires.Rght.Fx,VehFdbk.BdyFrm.Forces.Tires.RearTires.Lft.Fx,VehFdbk.BdyFrm.Forces.Tires.RearTires.Rght.Fx,VehFdbk.BdyFrm.Forces.Tires.FrntTires.Lft.Fy,VehFdbk.BdyFrm.Forces.Tires.FrntTires.Rght.Fy,VehFdbk.BdyFrm.Forces.Tires.RearTires.Lft.Fy,VehFdbk.BdyFrm.Forces.Tires.RearTires.Rght.Fy,VehFdbk.BdyFrm.Forces.Tires.FrntTires.Lft.Fz,VehFdbk.BdyFrm.Forces.Tires.FrntTires.Rght.Fz,VehFdbk.BdyFrm.Forces.Tires.RearTires.Lft.Fz,VehFdbk.BdyFrm.Forces.Tires.RearTires.Rght.Fz,VehFdbk.BdyFrm.Cg.Vel.xdot,VehFdbk.Mtr.MtrSpd,VehFdbk.Trans.TransGear
  Constant : Constant  Value="[[0.5100   -1.000    0.1000];[0.5100    1.000    0.1000];[-0.9900   -1.000    0.1000];[-0.9900    1.000    0.1000];[0.5100   -1.000    0.1000];[0.5100    1.000    0.1000];[-0.9900   -1.000    0.1000];[-0.9900    1.000    0.1000];[0.5100   -1.000    0.1000];[0.5100    1.000    0.1000];[-0.9900   -1.000    0.1000];-[0.9900]    1.000    0.1000]"
  Constant1 : Constant  Value=ones(3,1)
  Constant10 : Constant  Value=[zeros(3,1),[0.2;0.1;0],[2.5;2;1.5]]
  Constant2 : Constant  Value=logical(ones(3,1))
  Constant3 : Constant  Value=[zeros(3,1),[-0.7;-1.2;-0.7],[2.5;2;1.5]]
  Constant31 : Constant  Value=zeros(3,3)+[1 0 0]
  Constant32 : Constant  Value=zeros(3,3)
  Constant33 : Constant  Value=zeros(3,3)
  Constant4 : Constant  Value=ones(12,3)*1.8
  Constant5 : Constant  Value=[zeros(4,3)+[1 0 0]; zeros(4,3)+[0 1 0]; zeros(4,3)+[0 0 1]]
  Constant6 : Constant  Value=logical(ones(12,1))
  Constant7 : Constant  Value=zeros(3,3)+[1 0 0]
  Constant8 : Constant  Value=ones(3,1)
  Constant9 : Constant  Value=logical(ones(3,1))
  Convert to string : Subsystem
  Determine Angles In UE Vehicle Body Frame : Subsystem
  Forces : MATLABSystem  Priority=-1  System=Simulation3DAnnotation  InitialPos="[[0.5100   -1.000    0.1000];[0.5100    1.000    0.1000];[-0.9900   -1.000    0.1000];[-0.9900    1.000    0.1000];[0.5100   -1.000    0.1000];[0.5100    1.000    0.1000];[-0.9900   -1.000    0.1000];[-0.9900    1.000    0.1000];[0.5100   -1.000    0.1000];[0.5100    1.000    0.1000];[-0.9900   -1.000    0.1000];-[0.9900]    1.000    0.1000]"  InitialRot=[zeros(4,3);[zeros(4,3)+[0 0 pi/2]];[zeros(4,3)+[0 pi/2 0]]]  InitialScale=zeros(12,3)  ActorTag=AnnotationActor1  ParentActor=SimulinkVehicle1  Color=[zeros(4,3)+[1 0 0]; zeros(4,3)+[0 1 0]; zeros(4,3)+[0 0 1]]  Length=zeros(12,1)  FontScale=1  IsHidden=logical(zeros(12,1))  SampleTime=Ts
      mask Type: Simulation3DAnnotation
  Gain : Gain  Gain=[1 1 0 0].*pi/180*SteerLim
  Gain2 : Gain  Gain=1/500
  Labels : MATLABSystem  Priority=-1  System=Simulation3DAnnotation  InitialPos=[zeros(3,1),[-0.7;-0.7;-0.7],[2.5;2;1.5]]  InitialRot=zeros(3,3)  InitialScale=zeros(3,3)  ActorTag=AnnotationActor2  ParentActor=SimulinkVehicle1  Color=zeros(3,3)+[1 0 0]  Length=1  String=Velocity\n Motor (max)\n Gear  FontScale=ones(3,1)  IsHidden=logical(ones(3,1))  SampleTime=Ts
      mask Type: Simulation3DAnnotation
  Mux : Mux
  Mux1 : Mux
  Mux2 : Mux
  Stats : MATLABSystem  Priority=-1  System=Simulation3DAnnotation  InitialPos=[zeros(3,1),[0.2;0.1;0],[2.5;2;1.5]]  InitialRot=zeros(3,3)  InitialScale=zeros(3,3)  ActorTag=AnnotationActor3  ParentActor=SimulinkVehicle1  Color=zeros(3,3)+[1 0 0]  Length=1  String=00 km/h\n 0000 RPM\n 0  FontScale=ones(3,1)  IsHidden=logical(ones(3,1))  SampleTime=Ts
      mask Type: Simulation3DAnnotation
  String Constant : StringConstant  String="\"Velocity\\n Max Motor \\n Gear\""
  Vector Concatenate : Concatenate  NumInputs=3
  wires:
  VehFdbk/1 -> Bus Selector1/1
  Determine Angles In UE Vehicle Body Frame/1(Rotation) -> Forces/2
  Mux/1 -> Vector Concatenate/1, Determine Angles In UE Vehicle Body Frame/2(Fx)
  Mux1/1 -> Determine Angles In UE Vehicle Body Frame/3(Fy), Vector Concatenate/2
  Bus Selector1/1 -> Gain/1  "<SteerCmd>"
  Convert to string/1(String) -> Stats/4
  String Constant/1 -> Labels/4
  Constant33/1 -> Stats/2
  Constant31/1 -> Stats/3
  Constant8/1 -> Stats/5
  Constant9/1 -> Stats/6
  Constant32/1 -> Labels/2
  Constant3/1 -> Labels/1
  Constant7/1 -> Labels/3
  Constant1/1 -> Labels/5
  Constant2/1 -> Labels/6
  Constant10/1 -> Stats/1
  Constant/1 -> Forces/1
  Mux2/1 -> Vector Concatenate/3
  Abs/1 -> Gain2/1
  Vector Concatenate/1 -> Abs/1
  Gain2/1 -> Forces/5
  Constant4/1 -> Forces/3
  Constant6/1 -> Forces/6
  Constant5/1 -> Forces/4
  Gain/1 -> Determine Angles In UE Vehicle Body Frame/1(WheelYaw)
  Bus Selector1/2 -> Mux/1  "<Fx>"
  Bus Selector1/3 -> Mux/2  "<Fx>"
  Bus Selector1/4 -> Mux/3  "<Fx>"
  Bus Selector1/5 -> Mux/4  "<Fx>"
  Bus Selector1/6 -> Mux1/1  "<Fy>"
  Bus Selector1/7 -> Mux1/2  "<Fy>"
  Bus Selector1/8 -> Mux1/3  "<Fy>"
  Bus Selector1/9 -> Mux1/4  "<Fy>"
  Bus Selector1/10 -> Mux2/1  "<Fz>"
  Bus Selector1/11 -> Mux2/2  "<Fz>"
  Bus Selector1/12 -> Mux2/3  "<Fz>"
  Bus Selector1/13 -> Mux2/4  "<Fz>"
  Bus Selector1/14 -> Convert to string/1(xdot)  "<xdot>"
  Bus Selector1/15 -> Convert to string/2(MotorSpeed)  "<MtrSpd>"
  Bus Selector1/16 -> Convert to string/3(Gear)  "<TransGear>"

== system vdynblksskidpad_final/Visualization/3D Visualization/Enabled/3D Visualization/Simulation 3D Vehicle/Path/Disabled ==

== system vdynblksskidpad_final/Visualization/3D Visualization/Enabled/3D Visualization/Simulation 3D Vehicle/Path/Enabled ==
  VehFdbk : Inport
  Bus Selector : BusSelector  OutputSignals=VehFdbk.BdyFrm.Cg.Acc.ax,VehFdbk.BdyFrm.Cg.Acc.ay
  Constant5 : Constant
  Constant6 : Constant  Value=0
  Hypot : Math  Operator=hypot
  Saturation : Saturate  UpperLimit=1  LowerLimit=0  ZeroCross=off
  Simulation 3D Actor : sim3dlib/Simulation 3D Actor  Priority=10  ActorName=SimulinkPhysVehPath  ParentName=Scene Origin  Operation=Create at setup  InitScriptText=|  SampleTime=Ts*5  Translation=[0 0 0]  Rotation=[0 0 0]  Scale=[1 1 1]  InputsText=PathMarker.Color  aMode=5  ActorTag=SimulinkPhysVehPath  ActorType=Sim3dActor  ID=C
      | path1 = sim3d.graphics.PathMarker("ActorName", "PathMarker", ControlActorName="SimulinkVehicle1");
      | path1.MarkersSize = ones(1,3)*0.25;
      | path1.Color = [0 0 1];
      | World.add(path1,Actor);
  Sum1 : Sum  Inputs=|++
  Terminator4 : Terminator
  Unary Minus : UnaryMinus
  Vector Concatenate : Concatenate  NumInputs=3  Mode=Multidimensional array  ConcatenateDimension=2
  wires:
  Hypot/1 -> Saturation/1
  Saturation/1 -> Unary Minus/1, Vector Concatenate/1
  Constant5/1 -> Sum1/2
  Simulation 3D Actor/1 -> Terminator4/1
  Sum1/1 -> Vector Concatenate/3
  Unary Minus/1 -> Sum1/1
  Constant6/1 -> Vector Concatenate/2
  VehFdbk/1 -> Bus Selector/1
  Bus Selector/2 -> Hypot/2  "<ay>"
  Bus Selector/1 -> Hypot/1  "<ax>"
  Vector Concatenate/1 -> Simulation 3D Actor/1

== system vdynblksskidpad_final/Visualization/3D Visualization/Enabled/3D Visualization/Simulation 3D Vehicle/Scale/PartConcatenation ==
  BodyX : Inport
  BodyY : Inport  Port=2
  BodyZ : Inport  Port=3
  WheelFrontLeftX : Inport  Port=4
  WheelFrontLeftY : Inport  Port=5
  WheelFrontLeftZ : Inport  Port=6
  WheelFrontRightX : Inport  Port=7
  WheelFrontRightY : Inport  Port=8
  WheelFrontRightZ : Inport  Port=9
  WheelRearLeftX : Inport  Port=10
  WheelRearLeftY : Inport  Port=11
  WheelRearLeftZ : Inport  Port=12
  WheelRearRightX : Inport  Port=13
  WheelRearRightY : Inport  Port=14
  WheelRearRightZ : Inport  Port=15
  AllParts : Concatenate  NumInputs=5  Mode=Multidimensional array
  Body : Concatenate  NumInputs=3  Mode=Multidimensional array  ConcatenateDimension=2
  WheelFrontLeft : Concatenate  NumInputs=3  Mode=Multidimensional array  ConcatenateDimension=2
  WheelFrontRight : Concatenate  NumInputs=3  Mode=Multidimensional array  ConcatenateDimension=2
  WheelRearLeft : Concatenate  NumInputs=3  Mode=Multidimensional array  ConcatenateDimension=2
  WheelRearRight : Concatenate  NumInputs=3  Mode=Multidimensional array  ConcatenateDimension=2
  ConcatOut : Outport  VectorParamsAs1DForOutWhenUnconnected=off
  wires:
  BodyX/1 -> Body/1
  BodyZ/1 -> Body/3
  WheelFrontLeftX/1 -> WheelFrontLeft/1
  WheelFrontLeftZ/1 -> WheelFrontLeft/3
  WheelFrontLeftY/1 -> WheelFrontLeft/2
  BodyY/1 -> Body/2
  WheelFrontLeft/1 -> AllParts/2
  WheelRearRightX/1 -> WheelRearRight/1
  Body/1 -> AllParts/1
  WheelRearLeft/1 -> AllParts/4
  WheelFrontRight/1 -> AllParts/3
  WheelRearRightZ/1 -> WheelRearRight/3
  WheelFrontRightY/1 -> WheelFrontRight/2
  WheelFrontRightX/1 -> WheelFrontRight/1
  WheelRearRightY/1 -> WheelRearRight/2
  WheelRearLeftZ/1 -> WheelRearLeft/3
  AllParts/1 -> ConcatOut/1
  WheelRearLeftY/1 -> WheelRearLeft/2
  WheelRearRight/1 -> AllParts/5
  WheelRearLeftX/1 -> WheelRearLeft/1
  WheelFrontRightZ/1 -> WheelFrontRight/3

== system vdynblksskidpad_final/Visualization/3D Visualization/Enabled/3D Visualization/Ground Following/Annotations/Enabled/Convert to string ==
  xdot : Inport
  MotorSpeed : Inport  Port=2
  Gear : Inport  Port=3
  Round : Rounding  Operator=round
  Round1 : Rounding  Operator=round
  Signal Specification : SignalSpecification  Unit=rpm
  Signal Specification1 : SignalSpecification  Unit=km/h
  String Concatenate1 : StringConcatenate  Inputs=3
  String Concatenate2 : StringConcatenate
  String Concatenate3 : StringConcatenate
  String Constant3 : StringConstant  String="\" km/h\\n\""
  String Constant4 : StringConstant  String="\" RPM\\n\""
  To String1 : ToString
  To String2 : ToString
  To String3 : ToString
  Unit Conversion : UnitConversion
  Unit Conversion1 : UnitConversion
  String : Outport
  wires:
  MotorSpeed/1 -> Unit Conversion/1
  Signal Specification/1 -> Round1/1
  String Constant4/1 -> String Concatenate3/2
  Signal Specification1/1 -> Round/1
  String Concatenate2/1 -> String Concatenate1/1
  To String2/1 -> String Concatenate2/1
  String Constant3/1 -> String Concatenate2/2
  To String1/1 -> String Concatenate1/3
  String Concatenate3/1 -> String Concatenate1/2
  To String3/1 -> String Concatenate3/1
  Round/1 -> To String2/1
  Round1/1 -> To String3/1
  String Concatenate1/1 -> String/1
  Gear/1 -> To String1/1
  Unit Conversion/1 -> Signal Specification/1
  Unit Conversion1/1 -> Signal Specification1/1
  xdot/1 -> Unit Conversion1/1
